simulink model "Controlled_Single_Phase"  (R2025b)
settings: Solver=VariableStepAuto  StartTime=0.0  StopTime=10.0  RelTol=1e-3
libraries: nesl_utility x13, fl_lib x11, ee_lib x4
settings Model: Creator=USER  LastModifiedBy=USER

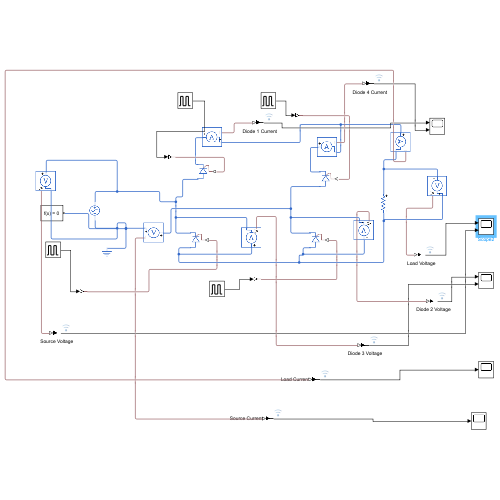
[thumbnail: Simulink's stored preview of the top-level diagram]
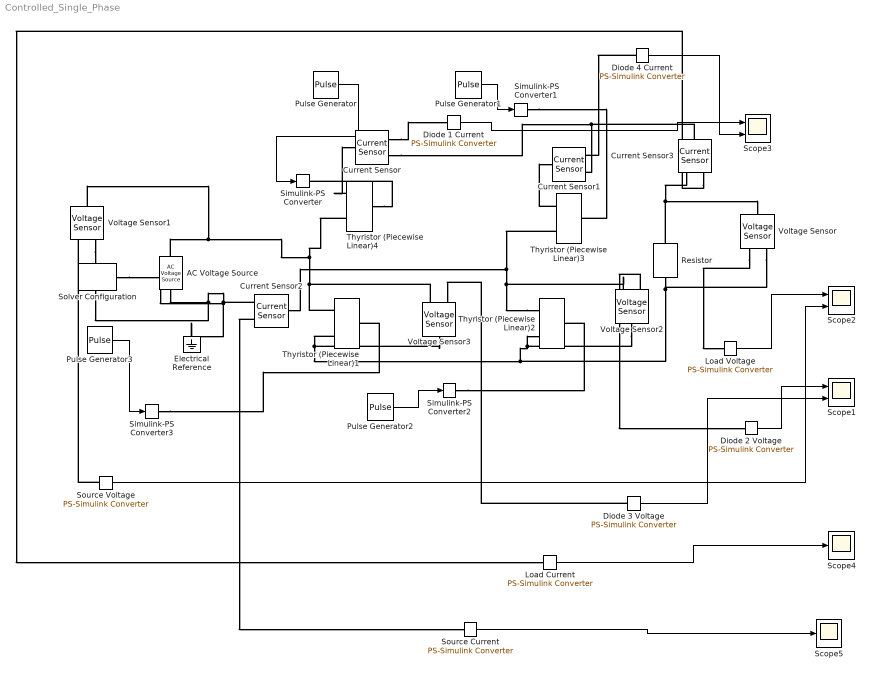
== system Controlled_Single_Phase ==
  AC Voltage Source : fl_lib/Electrical/Electrical Sources/AC Voltage Source  amp=127.28 V  shift=0 deg  frequency=50 Hz
  Current Sensor{,1..3} (4 alike) : fl_lib/Electrical/Electrical Sensors/Current Sensor
  Diode 1 Current : nesl_utility/PS-Simulink Converter  PhysicalDomain=network_engine_domain  SubClassName=ps_output  LeftPortType=input  RightPortType=output  PseudoPeriodic=off  Frequencies=[]  VectorFormat=inherit  Unit=inherit  AffineConversion=off
  Diode 2 Voltage : nesl_utility/PS-Simulink Converter  PhysicalDomain=network_engine_domain  SubClassName=ps_output  LeftPortType=input  RightPortType=output  PseudoPeriodic=off  Frequencies=[]  VectorFormat=inherit  Unit=inherit  AffineConversion=off
  Diode 3 Voltage : nesl_utility/PS-Simulink Converter  PhysicalDomain=network_engine_domain  SubClassName=ps_output  LeftPortType=input  RightPortType=output  PseudoPeriodic=off  Frequencies=[]  VectorFormat=inherit  Unit=inherit  AffineConversion=off
  Diode 4 Current : nesl_utility/PS-Simulink Converter  PhysicalDomain=network_engine_domain  SubClassName=ps_output  LeftPortType=input  RightPortType=output  PseudoPeriodic=off  Frequencies=[]  VectorFormat=inherit  Unit=inherit  AffineConversion=off
  Electrical Reference : fl_lib/Electrical/Electrical Elements/Electrical Reference
  Load Current : nesl_utility/PS-Simulink Converter  PhysicalDomain=network_engine_domain  SubClassName=ps_output  LeftPortType=input  RightPortType=output  PseudoPeriodic=off  Frequencies=[]  VectorFormat=inherit  Unit=inherit  AffineConversion=off
  Load Voltage : nesl_utility/PS-Simulink Converter  PhysicalDomain=network_engine_domain  SubClassName=ps_output  LeftPortType=input  RightPortType=output  PseudoPeriodic=off  Frequencies=[]  VectorFormat=inherit  Unit=inherit  AffineConversion=off
  Pulse Generator : DiscretePulseGenerator  PulseType=Time based  Amplitude=10  Period=0.02  PulseWidth=5  PhaseDelay=(30/360) * 0.02
  Pulse Generator1 : DiscretePulseGenerator  PulseType=Time based  Amplitude=10  Period=0.02  PulseWidth=5  PhaseDelay=(210/360) * 0.02
  Pulse Generator2 : DiscretePulseGenerator  PulseType=Time based  Amplitude=10  Period=0.02  PulseWidth=5  PhaseDelay=(30/360) * 0.02
  Pulse Generator3 : DiscretePulseGenerator  PulseType=Time based  Amplitude=10  Period=0.02  PulseWidth=5  PhaseDelay=(210/360) * 0.02
  Resistor : fl_lib/Electrical/Electrical Elements/Resistor  R=100 Ohm  i_specify=off  i_priority=None  i=0 A  i_nominal_specify=off  i_nominal_value=1  i_nominal_unit=A  v_specify=off  v_priority=None  v=0 V  v_nominal_specify=off  v_nominal_value=1  v_nominal_unit=V
  Scope1 : Scope  NumInputPorts=2
      settings: ActiveDisplayYMinimum=-146.1313884480287  ActiveDisplayYMaximum=50.395647763876724
  Scope2 : Scope  NumInputPorts=2
      settings: ActiveDisplayYMinimum=-133.8163626727231  ActiveDisplayYMaximum=184.38363732727876  DataLoggingVariableName=ScopeData2
  Scope3 : Scope  NumInputPorts=2
      settings: ActiveDisplayYMinimum=-0.15867246450836542  ActiveDisplayYMaximum=1.4154047321004675
  Scope4 : Scope
      settings: ActiveDisplayYMinimum=-1.5740135626199416  ActiveDisplayYMaximum=1.5740701261655559  DataLoggingVariableName=ScopeData3
  Scope5 : Scope
      settings: ActiveDisplayYMinimum=-1.7186498537713666  ActiveDisplayYMaximum=1.4294338350141309  DataLoggingVariableName=ScopeData4
  Simulink-PS Converter{,1..3} (4 alike) : nesl_utility/Simulink-PS Converter  PhysicalDomain=network_engine_domain  SubClassName=ps_input  LeftPortType=input  RightPortType=output  PseudoPeriodic=off  Frequencies=[]  NoiseDistribution=none  NoiseParameters=[]  Unit=1  AffineConversion=off  FilteringAndDerivatives=provide  SimscapeFilterOrder=1  InputFilterTimeConstant=0.001  UdotUserProvided=0
  Solver Configuration : nesl_utility/Solver Configuration  PhysicalDomain=network_engine_domain  SubClassName=solver  LeftPortType=input  RightPortType=generic  Tones=[]  Harmonics=[]  SimulateNoise=off  Profile=off  UseLocalSampling=off  EnableSwitchedLinearOptims=on  FrequencyDomain=off  UseCCode=off  RelTol=0.001  AbsTol=0.001  MinStep=1e-09  ToWorkspace=off  RevertToSquareIcSolve=off  NumHomotopyIterations=100  PhasorMode=off  PhasorModeNumHarmonics=1  ConsistencySolver=NEWTON_XTOL_AFTER_FTOL  IndexReductionMethod=DerivativeReplacement  DoDC=off  ResidualTolerance=1e-09  ConsistencyTolSource=GLOBAL  ConsistencyAbsTol=0.001  ConsistencyRelTol=0.001  ConsistencyTolFactor=0.001  UseLocalSolver=off  LocalSolverChoice=NE_BACKWARD_EULER_ADVANCER  ResolveIndetEquations=on  FunctionEvalNumThread=1  LocalSolverSampleTime=0.001  DoFixedCost=off  MaxNonlinIter=3  MaxModeIter=2  ComputeImpulses=off  ImpulseIterations=2  LinearAlgebra=auto  LinearAlgebraNumThread=0  EquationFormulation=NE_TIME_EF  DelaysMemoryBudget=1024  AutomaticFiltering=on  FilteringTimeConstant=0.001  PartitionStorageMethod=AS_NEEDED  PartitionMemoryBudget=1024  PartitionMethod=ROBUST  MultibodyUseLocalSolver=off  MultibodyLocalSolverChoice=ODE1  MultibodyLocalSolverSampleTime=0.001
  Source Current : nesl_utility/PS-Simulink Converter  PhysicalDomain=network_engine_domain  SubClassName=ps_output  LeftPortType=input  RightPortType=output  PseudoPeriodic=off  Frequencies=[]  VectorFormat=inherit  Unit=inherit  AffineConversion=off
  Source Voltage : nesl_utility/PS-Simulink Converter  PhysicalDomain=network_engine_domain  SubClassName=ps_output  LeftPortType=input  RightPortType=output  PseudoPeriodic=off  Frequencies=[]  VectorFormat=inherit  Unit=inherit  AffineConversion=off
  Thyristor (Piecewise Linear){1..4} (4 alike) : ee_lib/Semiconductors & Converters/Thyristor (Piecewise Linear)  port_option=ee.enum.controlport.ps  Vf=0.8 V  Ron=0.001 Ohm  Goff=1e-5 1/Ohm  Vgt=6 V  Ih=0.1 A  diode_param=ee.enum.semiconductors.protectionDiode.external  diode_Vf=0.8 V  diode_Ron=0.001 Ohm  diode_Goff=1e-5 1/Ohm  diode_C=50e-9 F  diode_iRM=-235 A  diode_iF=300 A  diode_idot=-50 A/us  diode_trr_param=ee.enum.converters.diodetrr.trr_factor  diode_trr_factor=3  diode_trr=15 us  diode_Qrr=1500 s*uA  iak_specify=off  iak_priority=None  iak=0 A  iak_nominal_specify=off  iak_nominal_value=1  iak_nominal_unit=A  vak_specify=off  vak_priority=None  vak=0 V  vak_nominal_specify=off  vak_nominal_value=1  vak_nominal_unit=V  vgk_specify=off  vgk_priority=None  vgk=0 V  vgk_nominal_specify=off  vgk_nominal_value=1  vgk_nominal_unit=V  thermal_loss_option=ee.enum.converters.thermalLossOption.constantvalues  Von_data=[0, .1, .6, .8, 1, 1.3, 1.6, 2, 2.4; 0, .1, .7, 1, 1.2, 1.5, 1.9, 2.4, 2.8] V  Tj=[298.15, 398.15] K  Iout_data=[0, .1, 1, 5, 10, 20, 40, 70, 100] A  Eon_data=[0, .0024, .024, .12, .2, .48, 1.04, 2.16, 3.24; 0, .003, .03, .15, .25, .6, 1.3, 2.7, 4.05] * 1e-3 J  Tj_loss=[298.15, 398.15] K  Iout_data_loss=[0, .1, 1, 5, 10, 20, 40, 70, 100] A  Eon_scalar=22.86e-3 J  Eoff_natural_commutation=10e-3 J  Voff=300 V  Iout_scalar=600 A  onCurrentMeasDelay=1e-4 s  diodeModelType=ee.enum.converters.diodeModelType.pwl  diodeTableType=ee.enum.diode.tableType.IfMat  diode_IfMat=[.07, .12, .19, 1.75, 4.24, 7.32, 11.2; .16, .3, .72, 2.14, 4.02, 6.35, 9.12] A  diode_VfMat=[.9, 1.15, 1.25, 1.5, 1.75, 2.17, 2.6, 2.85; .58, .68, .75, 1.1, 1.38, 1.77, 2.27, 2.7] V  diode_TjVec=[25, 125] degC  diode_VfVec=[.5, .7, .9, 1.3, 1.7, 2.1, 2.5] V  diode_IfVec=[.1, .2, .5, 1, 2, 4, 7, 10] A  diode_rec_loss_model=ee.enum.diode.reverseRecoveryModel.fixed  diode_ErecVal=0 J  diode_scaleWithIandV=true  diode_ErecMat=zeros(2, 3) J  diode_TjrecVec=[298.15, 398.15] K  diode_IfrecVec=[.1, 1, 10] A  diode_IrecVal=10 A  diode_VrecVal=10 V  diode_tFilter=1 / 1000 / 100 s  thermal_network_parameterization=ee.enum.thermalNetworkTopology.external  Rth=[.08, .5] K/W  Rth_Cauer=[.08, .1, .5] K/W  Rth_Foster=[.08, .14, .22, .16] K/W  thermal_mass_parameterization=ee.enum.thermalNetwork.timeconstant  thermal_mass=[.01, .5] J/K  thermal_mass_Cauer=[.01, .1, .5] J/K  thermal_mass_Foster=[.001, .005, .05, .5] J/K  thermal_time_constant=[.001, .2] s  thermal_time_constant_Cauer=[.001, .1, .2] s  thermal_time_constant_Foster=[7e-05, .0007, .01, .08] s  thermal_mass_initial_temperatures=[25, 25] degC  thermal_mass_initial_temperatures_Cauer=[25, 25, 25] degC  junction_thermal_mass=0.01 J/K  Tvec_initial_Foster=[25, 25, 25, 25] degC  junction_temperature_specify=off  junction_temperature_priority=None  junction_temperature=25 degC  junction_temperature_nominal_specify=off  junction_temperature_nominal_value=1  junction_temperature_nominal_unit=degC  Qj_specify=off  Qj_priority=None  Qj=0 W  Qj_nominal_specify=off  Qj_nominal_value=1  Qj_nominal_unit=W  accumulatedSwitchingLosses_specify=off  accumulatedSwitchingLosses_priority=None  accumulatedSwitchingLosses=0 J
      settings: InternalSimscapePortConfiguration="{\"Bottom\":[],\"Left\":[{\"id\":\"G\",\"label\":\"\",\"type\":\"input\"}],\"Right\":[{\"id\":\"A\",\"label\":\"\",\"type\":\"foundation.electrical.electrical\"},{\"id\":\"K\",\"label\":\"\",\"type\":\"foundation.electrical.electrical\"}],\"Top\":[]}"
  Voltage Sensor{,1..3} (4 alike) : fl_lib/Electrical/Electrical Sensors/Voltage Sensor
  wires:
  Pulse Generator/1 -> Simulink-PS Converter/1
  Pulse Generator1/1 -> Simulink-PS Converter1/1
  Pulse Generator2/1 -> Simulink-PS Converter2/1
  Pulse Generator3/1 -> Simulink-PS Converter3/1
  Load Voltage/1 -> Scope2/1
  Source Voltage/1 -> Scope2/2
  Diode 2 Voltage/1 -> Scope1/1
  Diode 3 Voltage/1 -> Scope1/2
  Diode 1 Current/1 -> Scope3/1
  Diode 4 Current/1 -> Scope3/2
  Source Current/1 -> Scope5/1
  Load Current/1 -> Scope4/1
  connections:
  Thyristor (Piecewise Linear)4/RConn1 -- AC Voltage Source/LConn1 -- Voltage Sensor1/LConn1 -- Voltage Sensor3/RConn2 -- Thyristor (Piecewise Linear)1/RConn2
  Resistor/LConn1 -- Voltage Sensor/LConn1 -- Current Sensor3/RConn2
  Thyristor (Piecewise Linear)1/RConn1 -- Voltage Sensor3/LConn1 -- Voltage Sensor/RConn2 -- Resistor/RConn1 -- Voltage Sensor2/LConn1 -- Thyristor (Piecewise Linear)2/RConn1
  AC Voltage Source/RConn1 -- Voltage Sensor1/RConn2 -- Electrical Reference/LConn1 -- Solver Configuration/RConn1 -- Current Sensor2/RConn2
  Simulink-PS Converter1/RConn1 -- Thyristor (Piecewise Linear)3/LConn1
  Simulink-PS Converter2/RConn1 -- Thyristor (Piecewise Linear)2/LConn1
  Simulink-PS Converter3/RConn1 -- Thyristor (Piecewise Linear)1/LConn1
  Voltage Sensor/RConn1 -- Load Voltage/LConn1
  Source Voltage/LConn1 -- Voltage Sensor1/RConn1
  Voltage Sensor2/RConn1 -- Diode 2 Voltage/LConn1
  Diode 3 Voltage/LConn1 -- Voltage Sensor3/RConn1
  Thyristor (Piecewise Linear)4/LConn1 -- Simulink-PS Converter/RConn1
  Thyristor (Piecewise Linear)4/RConn2 -- Current Sensor/LConn1
  Current Sensor/RConn1 -- Diode 1 Current/LConn1
  Thyristor (Piecewise Linear)3/RConn2 -- Current Sensor1/LConn1
  Diode 4 Current/LConn1 -- Current Sensor1/RConn1
  Current Sensor2/RConn1 -- Source Current/LConn1
  Current Sensor/RConn2 -- Current Sensor3/LConn1 -- Current Sensor1/RConn2
  Current Sensor3/RConn1 -- Load Current/LConn1
  Thyristor (Piecewise Linear)2/RConn2 -- Current Sensor2/LConn1 -- Thyristor (Piecewise Linear)3/RConn1 -- Voltage Sensor2/RConn2
